simulink model "rolling_contact_36_example"  (R2026b)
settings: Solver=VariableStepAuto  StopTime=5
undefined symbols (not defined in the file): f_rr, k_gx, k_gy, k_x, m_wheel, miu_p, miu_s, mu_slide, mu_stick, omega_rr_eps, r_wheel, sgn, v_gx_max, v_gy_max, vLimit, X, Y, Z
libraries: nesl_utility x225, sm_lib x156, simulink x146, simulink_extras x36
(part 6 of 11)

== system rolling_contact_36_example/36-Point Sliding Contact Model/Body Contact 8 ==
  note: Planar Ground Interaction Model
  " Body Actuator" : nesl_utility/Simulink-PS Converter  PhysicalDomain=network_engine_domain  SubClassName=ps_input  LeftPortType=input  RightPortType=output  PseudoPeriodic=off  Frequencies=[]  NoiseDistribution=none  NoiseParameters=[]  Unit=N  AffineConversion=off  FilteringAndDerivatives=zero  SimscapeFilterOrder=1  InputFilterTimeConstant=.001  UdotUserProvided=0
  " Body Actuator1" : nesl_utility/Simulink-PS Converter  PhysicalDomain=network_engine_domain  SubClassName=ps_input  LeftPortType=input  RightPortType=output  PseudoPeriodic=off  Frequencies=[]  NoiseDistribution=none  NoiseParameters=[]  Unit=N  AffineConversion=off  FilteringAndDerivatives=zero  SimscapeFilterOrder=1  InputFilterTimeConstant=.001  UdotUserProvided=0
  External Force and Torque : sm_lib/Forces and Torques/External Force and Torque  EnableForceX=on  EnableForceY=on  EnableForceZ=off  EnableForce=off  ForceResolutionFrame=World  EnableTorqueX=off  EnableTorqueY=off  EnableTorqueZ=off  EnableTorque=off  TorqueResolutionFrame=AttachedFrame
  Frame Sensor : sm_lib/Frames and Transforms/Transform Sensor  ObservationFrame=World  ExpressedInFrame=World  RotationSequence=XYX  SenseAngle=off  SenseAxis=off  SenseQ=off  SenseR=off  SenseRotationSequence=off  SenseOmegaX=off  SenseOmegaY=off  SenseOmegaZ=off  SenseOmega=off  SenseQDot=off  SenseRDot=off  SenseRotationSequenceDot=off  SenseAlphaX=off  SenseAlphaY=off  SenseAlphaZ=off  SenseAlpha=off  SenseQDDot=off  SenseRDDot=off  SenseX=on  SenseY=on  SenseZ=off  SenseXYZ=off  SenseRad=off  SenseAzim=off  SenseDist=off  SenseInc=off  SenseXDot=on  SenseYDot=on  SenseZDot=off  SenseXYZDot=off  SenseRadDot=off  SenseAzimDot=off  SenseDistDot=off  SenseIncDot=off  SenseXDDot=off  SenseYDDot=off  SenseZDDot=off  SenseXYZDDot=off  SenseRadDDot=off  SenseAzimDDot=off  SenseDistDDot=off  SenseIncDDot=off
  Ground Friction Model : Subsystem
  PS-Simulink Converter : nesl_utility/PS-Simulink Converter  PhysicalDomain=network_engine_domain  SubClassName=ps_output  LeftPortType=input  RightPortType=output  PseudoPeriodic=off  Frequencies=[]  VectorFormat=1-D array  Unit=m  AffineConversion=off
  PS-Simulink Converter1 : nesl_utility/PS-Simulink Converter  PhysicalDomain=network_engine_domain  SubClassName=ps_output  LeftPortType=input  RightPortType=output  PseudoPeriodic=off  Frequencies=[]  VectorFormat=1-D array  Unit=m  AffineConversion=off
  PS-Simulink Converter2 : nesl_utility/PS-Simulink Converter  PhysicalDomain=network_engine_domain  SubClassName=ps_output  LeftPortType=input  RightPortType=output  PseudoPeriodic=off  Frequencies=[]  VectorFormat=1-D array  Unit=m/s  AffineConversion=off
  PS-Simulink Converter3 : nesl_utility/PS-Simulink Converter  PhysicalDomain=network_engine_domain  SubClassName=ps_output  LeftPortType=input  RightPortType=output  PseudoPeriodic=off  Frequencies=[]  VectorFormat=1-D array  Unit=m/s  AffineConversion=off
  Sum : Sum  Inputs=-+|
  Terminator : Terminator
  World Frame : sm_lib/Frames and Transforms/World Frame
  contact sensor : simulink/Logic and Bit Operations/Compare To Zero  relop=<=  OutDataTypeStr=boolean
  yGround : Constant  Value=0
  F : PMIOPort  Side=Left
  Fx patch [N] : Outport
  Fy patch [N] : Outport  Port=2
  wires:
  Ground Friction Model/3(Stiction!) -> Terminator/1
  Ground Friction Model/2(Fx_Friction [N]) -> " Body Actuator"/1, Fx patch [N]/1
  Ground Friction Model/1(Fy_Ground[N]) -> " Body Actuator1"/1, Fy patch [N]/1
  contact sensor/1 -> Ground Friction Model/Enable
  yGround/1 -> Sum/1
  Sum/1 -> Ground Friction Model/1(dy [m]), contact sensor/1
  PS-Simulink Converter1/1 -> Sum/2
  PS-Simulink Converter3/1 -> Ground Friction Model/2(vy [m/s])
  PS-Simulink Converter/1 -> Ground Friction Model/3(x [m])
  PS-Simulink Converter2/1 -> Ground Friction Model/4(vx [m/s])
  connections:
  External Force and Torque/LConn1 -- " Body Actuator"/RConn1
  External Force and Torque/LConn2 -- " Body Actuator1"/RConn1
  F/RConn1 -- Frame Sensor/RConn1 -- External Force and Torque/RConn1
  PS-Simulink Converter3/LConn1 -- Frame Sensor/RConn5
  Frame Sensor/RConn2 -- PS-Simulink Converter/LConn1
  PS-Simulink Converter1/LConn1 -- Frame Sensor/RConn3
  PS-Simulink Converter2/LConn1 -- Frame Sensor/RConn4
  World Frame/RConn1 -- Frame Sensor/LConn1

== system rolling_contact_36_example/36-Point Sliding Contact Model/Body Contact 9 ==
  note: Planar Ground Interaction Model
  " Body Actuator" : nesl_utility/Simulink-PS Converter  PhysicalDomain=network_engine_domain  SubClassName=ps_input  LeftPortType=input  RightPortType=output  PseudoPeriodic=off  Frequencies=[]  NoiseDistribution=none  NoiseParameters=[]  Unit=N  AffineConversion=off  FilteringAndDerivatives=zero  SimscapeFilterOrder=1  InputFilterTimeConstant=.001  UdotUserProvided=0
  " Body Actuator1" : nesl_utility/Simulink-PS Converter  PhysicalDomain=network_engine_domain  SubClassName=ps_input  LeftPortType=input  RightPortType=output  PseudoPeriodic=off  Frequencies=[]  NoiseDistribution=none  NoiseParameters=[]  Unit=N  AffineConversion=off  FilteringAndDerivatives=zero  SimscapeFilterOrder=1  InputFilterTimeConstant=.001  UdotUserProvided=0
  External Force and Torque : sm_lib/Forces and Torques/External Force and Torque  EnableForceX=on  EnableForceY=on  EnableForceZ=off  EnableForce=off  ForceResolutionFrame=World  EnableTorqueX=off  EnableTorqueY=off  EnableTorqueZ=off  EnableTorque=off  TorqueResolutionFrame=AttachedFrame
  Frame Sensor : sm_lib/Frames and Transforms/Transform Sensor  ObservationFrame=World  ExpressedInFrame=World  RotationSequence=XYX  SenseAngle=off  SenseAxis=off  SenseQ=off  SenseR=off  SenseRotationSequence=off  SenseOmegaX=off  SenseOmegaY=off  SenseOmegaZ=off  SenseOmega=off  SenseQDot=off  SenseRDot=off  SenseRotationSequenceDot=off  SenseAlphaX=off  SenseAlphaY=off  SenseAlphaZ=off  SenseAlpha=off  SenseQDDot=off  SenseRDDot=off  SenseX=on  SenseY=on  SenseZ=off  SenseXYZ=off  SenseRad=off  SenseAzim=off  SenseDist=off  SenseInc=off  SenseXDot=on  SenseYDot=on  SenseZDot=off  SenseXYZDot=off  SenseRadDot=off  SenseAzimDot=off  SenseDistDot=off  SenseIncDot=off  SenseXDDot=off  SenseYDDot=off  SenseZDDot=off  SenseXYZDDot=off  SenseRadDDot=off  SenseAzimDDot=off  SenseDistDDot=off  SenseIncDDot=off
  Ground Friction Model : Subsystem
  PS-Simulink Converter : nesl_utility/PS-Simulink Converter  PhysicalDomain=network_engine_domain  SubClassName=ps_output  LeftPortType=input  RightPortType=output  PseudoPeriodic=off  Frequencies=[]  VectorFormat=1-D array  Unit=m  AffineConversion=off
  PS-Simulink Converter1 : nesl_utility/PS-Simulink Converter  PhysicalDomain=network_engine_domain  SubClassName=ps_output  LeftPortType=input  RightPortType=output  PseudoPeriodic=off  Frequencies=[]  VectorFormat=1-D array  Unit=m  AffineConversion=off
  PS-Simulink Converter2 : nesl_utility/PS-Simulink Converter  PhysicalDomain=network_engine_domain  SubClassName=ps_output  LeftPortType=input  RightPortType=output  PseudoPeriodic=off  Frequencies=[]  VectorFormat=1-D array  Unit=m/s  AffineConversion=off
  PS-Simulink Converter3 : nesl_utility/PS-Simulink Converter  PhysicalDomain=network_engine_domain  SubClassName=ps_output  LeftPortType=input  RightPortType=output  PseudoPeriodic=off  Frequencies=[]  VectorFormat=1-D array  Unit=m/s  AffineConversion=off
  Sum : Sum  Inputs=-+|
  Terminator : Terminator
  World Frame : sm_lib/Frames and Transforms/World Frame
  contact sensor : simulink/Logic and Bit Operations/Compare To Zero  relop=<=  OutDataTypeStr=boolean
  yGround : Constant  Value=0
  F : PMIOPort  Side=Left
  Fx patch [N] : Outport
  Fy patch [N] : Outport  Port=2
  wires:
  PS-Simulink Converter2/1 -> Ground Friction Model/4(vx [m/s])
  PS-Simulink Converter/1 -> Ground Friction Model/3(x [m])
  PS-Simulink Converter3/1 -> Ground Friction Model/2(vy [m/s])
  PS-Simulink Converter1/1 -> Sum/2
  Sum/1 -> contact sensor/1, Ground Friction Model/1(dy [m])
  yGround/1 -> Sum/1
  contact sensor/1 -> Ground Friction Model/Enable
  Ground Friction Model/1(Fy_Ground[N]) -> " Body Actuator1"/1, Fy patch [N]/1
  Ground Friction Model/2(Fx_Friction [N]) -> " Body Actuator"/1, Fx patch [N]/1
  Ground Friction Model/3(Stiction!) -> Terminator/1
  connections:
  World Frame/RConn1 -- Frame Sensor/LConn1
  PS-Simulink Converter2/LConn1 -- Frame Sensor/RConn4
  PS-Simulink Converter1/LConn1 -- Frame Sensor/RConn3
  Frame Sensor/RConn2 -- PS-Simulink Converter/LConn1
  PS-Simulink Converter3/LConn1 -- Frame Sensor/RConn5
  External Force and Torque/RConn1 -- Frame Sensor/RConn1 -- F/RConn1
  External Force and Torque/LConn2 -- " Body Actuator1"/RConn1
  External Force and Torque/LConn1 -- " Body Actuator"/RConn1

== system rolling_contact_36_example/Rolling Contact Model/Rolling Resistance Model ==
  Fy [N] : Inport
  wheel speed [rad/s] : Inport  Port=2
  Contact! : EnablePort
  Input Mux : Mux  Inputs=2
  Rolling Resistance Law : Fcn  Expr=-f_rr * u(2) * r_wheel * tanh(u(1) / omega_rr_eps)
  tau_rr [N*m] : Outport
  wires:
  wheel speed [rad/s]/1 -> Input Mux/1
  Fy [N]/1 -> Input Mux/2
  Rolling Resistance Law/1 -> tau_rr [N*m]/1
  Input Mux/1 -> Rolling Resistance Law/1

== system rolling_contact_36_example/Rolling Contact Model/Slip Resistance Model ==
  note: Normal Contact Force
  note: Slip Resistance Force
  note: Peak Slip Ratio (lambda*)
  dy [m] : Inport
  vy [m/s] : Inport  Port=2
  slip ratio : Inport  Port=3
  Contact! : EnablePort  StatesWhenEnabling=reset
  Characteristic Slip Ratio : Fcn  Expr=(3 * miu_p * u(2))/(2 * (u(1)^2 + 0.000000000001) * k_x)
  Constant : Constant  Value=k_x
  Constant1 : Constant  Value=miu_p
  Constant2 : Constant  Value=miu_s
  Gain : Gain  Gain=-r_wheel
  Gain3 : Gain  Gain=pi/4 * E * 1
  Gain4 : Gain  Gain=1/v_gy_max
  Longitudinal Brush Force : MATLAB Function  TreatAsAtomicUnit=on
  Mux : Mux  Inputs=2
  Mux1 : Mux  Inputs=2
  Sqrt : Sqrt
  Y-Axis Ground Force : Fcn  Expr=- u(1) * (1-u(2)) * (u(2)<1)
  Fy_Ground[N] : Outport  OutputWhenDisabled=reset  InitialOutput=0
      settings: AttributesFormatString=initial = '%<InitialOutput>'\nwhen disabled = '%<OutputWhenDisabled>'
  Fx_Friction [N] : Outport  Port=2  OutputWhenDisabled=reset  InitialOutput=0
      settings: AttributesFormatString=initial = '%<InitialOutput>'\nwhen\ndisabled\n'%<OutputWhenDisabled>'
  wires:
  Gain4/1 -> Mux/2
  dy [m]/1 -> Gain3/1, Gain/1  "displacement"
  Mux/1 -> Y-Axis Ground Force/1
  vy [m/s]/1 -> Gain4/1
  Gain3/1 -> Mux/1
  Gain/1 -> Sqrt/1
  Sqrt/1 -> Longitudinal Brush Force/3(a), Mux1/1  "1/2 contact width (a)"
  Mux1/1 -> Characteristic Slip Ratio/1
  Y-Axis Ground Force/1 -> Fy_Ground[N]/1, Longitudinal Brush Force/4(Fy), Mux1/2
  slip ratio/1 -> Longitudinal Brush Force/1(lamda)
  Characteristic Slip Ratio/1 -> Longitudinal Brush Force/2(lamda_c)
  Constant/1 -> Longitudinal Brush Force/5(k_x)
  Constant1/1 -> Longitudinal Brush Force/6(miu_p)
  Constant2/1 -> Longitudinal Brush Force/7(miu_s)
  Longitudinal Brush Force/1(y) -> Fx_Friction [N]/1

== system rolling_contact_36_example/36-Point Sliding Contact Model/Body Contact /Ground Friction Model ==
  note: Vertical Ground Stiction Model
  note: Horizontal Ground Friction Model
  dy [m] : Inport
  vy [m/s] : Inport  Port=2
  x [m] : Inport  Port=3
  vx [m/s] : Inport  Port=4
  Contact! : EnablePort  StatesWhenEnabling=reset
  Data Type Conversion : DataTypeConversion  OutDataTypeStr=double  SaturateOnIntegerOverflow=off  RndMeth=Floor
  Friction Switch : Subsystem
  Gain3 : Gain  Gain=k_gy
  Gain4 : Gain  Gain=1/v_gy_max
  Logical Operator : Logic  Operator=NOT  AllPortsSameDT=off  OutDataTypeStr=boolean
  Mux1 : Mux  Inputs=2
  Sum1 : Sum
  X-Axis Kinetic Friction Model : Subsystem
  X-Axis Static Friction Model : Subsystem
  Y-Axis Ground Force : Fcn  Expr="- u(1)  *  (1-u(2)) * (u(2)<1)"
  Fy_Ground[N] : Outport  OutputWhenDisabled=reset  InitialOutput=0
      settings: AttributesFormatString=initial = '%<InitialOutput>'\nwhen disabled = '%<OutputWhenDisabled>'
  Fx_Friction [N] : Outport  Port=2  OutputWhenDisabled=reset  InitialOutput=0
      settings: AttributesFormatString=initial = '%<InitialOutput>'\nwhen\ndisabled\n'%<OutputWhenDisabled>'
  Stiction! : Outport  Port=3  OutputWhenDisabled=reset  InitialOutput=0
      settings: AttributesFormatString=initial = '%<InitialOutput>'\nwhen\ndisabled\n'%<OutputWhenDisabled>'
  wires:
  Gain4/1 -> Mux1/2
  Gain3/1 -> Mux1/1
  Mux1/1 -> Y-Axis Ground Force/1
  Data Type Conversion/1 -> Stiction!/1
  Logical Operator/1 -> X-Axis Kinetic Friction Model/Enable
  X-Axis Kinetic Friction Model/2(Stiction!) -> Friction Switch/2(Stick!)
  X-Axis Static Friction Model/2(Sliding!) -> Friction Switch/1(Slide!)
  Friction Switch/1(Stiction) -> Data Type Conversion/1, Logical Operator/1, X-Axis Static Friction Model/Enable
  Sum1/1 -> Fx_Friction [N]/1
  X-Axis Static Friction Model/1(F_Stick [N]) -> Sum1/1
  X-Axis Kinetic Friction Model/3(F_Slide [N]) -> Sum1/2
  X-Axis Kinetic Friction Model/1(posFP [m]) -> X-Axis Static Friction Model/4(posFP [m])
  vx [m/s]/1 -> X-Axis Kinetic Friction Model/2(vel [m/s]), X-Axis Static Friction Model/3(vel [m/s])
  x [m]/1 -> X-Axis Kinetic Friction Model/1(pos [m]), X-Axis Static Friction Model/2(pos [m])
  vy [m/s]/1 -> Gain4/1
  dy [m]/1 -> Gain3/1
  Y-Axis Ground Force/1 -> Fy_Ground[N]/1, X-Axis Kinetic Friction Model/3(F_Normal [N]), X-Axis Static Friction Model/1(F_Normal [N])

== system rolling_contact_36_example/36-Point Sliding Contact Model/Body Contact 1/Ground Friction Model ==
  note: Horizontal Ground Friction Model
  note: Vertical Ground Stiction Model
  dy [m] : Inport
  vy [m/s] : Inport  Port=2
  x [m] : Inport  Port=3
  vx [m/s] : Inport  Port=4
  Contact! : EnablePort  StatesWhenEnabling=reset
  Data Type Conversion : DataTypeConversion  OutDataTypeStr=double  SaturateOnIntegerOverflow=off  RndMeth=Floor
  Friction Switch : Subsystem
  Gain3 : Gain  Gain=k_gy
  Gain4 : Gain  Gain=1/v_gy_max
  Logical Operator : Logic  Operator=NOT  AllPortsSameDT=off  OutDataTypeStr=boolean
  Mux1 : Mux  Inputs=2
  Sum1 : Sum
  X-Axis Kinetic Friction Model : Subsystem
  X-Axis Static Friction Model : Subsystem
  Y-Axis Ground Force : Fcn  Expr="- u(1)  *  (1-u(2)) * (u(2)<1)"
  Fy_Ground[N] : Outport  OutputWhenDisabled=reset  InitialOutput=0
      settings: AttributesFormatString=initial = '%<InitialOutput>'\nwhen disabled = '%<OutputWhenDisabled>'
  Fx_Friction [N] : Outport  Port=2  OutputWhenDisabled=reset  InitialOutput=0
      settings: AttributesFormatString=initial = '%<InitialOutput>'\nwhen\ndisabled\n'%<OutputWhenDisabled>'
  Stiction! : Outport  Port=3  OutputWhenDisabled=reset  InitialOutput=0
      settings: AttributesFormatString=initial = '%<InitialOutput>'\nwhen\ndisabled\n'%<OutputWhenDisabled>'
  wires:
  Y-Axis Ground Force/1 -> X-Axis Static Friction Model/1(F_Normal [N]), X-Axis Kinetic Friction Model/3(F_Normal [N]), Fy_Ground[N]/1
  dy [m]/1 -> Gain3/1
  vy [m/s]/1 -> Gain4/1
  x [m]/1 -> X-Axis Static Friction Model/2(pos [m]), X-Axis Kinetic Friction Model/1(pos [m])
  vx [m/s]/1 -> X-Axis Static Friction Model/3(vel [m/s]), X-Axis Kinetic Friction Model/2(vel [m/s])
  X-Axis Kinetic Friction Model/1(posFP [m]) -> X-Axis Static Friction Model/4(posFP [m])
  X-Axis Kinetic Friction Model/3(F_Slide [N]) -> Sum1/2
  X-Axis Static Friction Model/1(F_Stick [N]) -> Sum1/1
  Sum1/1 -> Fx_Friction [N]/1
  Friction Switch/1(Stiction) -> X-Axis Static Friction Model/Enable, Logical Operator/1, Data Type Conversion/1
  X-Axis Static Friction Model/2(Sliding!) -> Friction Switch/1(Slide!)
  X-Axis Kinetic Friction Model/2(Stiction!) -> Friction Switch/2(Stick!)
  Logical Operator/1 -> X-Axis Kinetic Friction Model/Enable
  Data Type Conversion/1 -> Stiction!/1
  Mux1/1 -> Y-Axis Ground Force/1
  Gain3/1 -> Mux1/1
  Gain4/1 -> Mux1/2

== system rolling_contact_36_example/36-Point Sliding Contact Model/Body Contact 10/Ground Friction Model ==
  note: Vertical Ground Stiction Model
  note: Horizontal Ground Friction Model
  dy [m] : Inport
  vy [m/s] : Inport  Port=2
  x [m] : Inport  Port=3
  vx [m/s] : Inport  Port=4
  Contact! : EnablePort  StatesWhenEnabling=reset
  Data Type Conversion : DataTypeConversion  OutDataTypeStr=double  SaturateOnIntegerOverflow=off  RndMeth=Floor
  Friction Switch : Subsystem
  Gain3 : Gain  Gain=k_gy
  Gain4 : Gain  Gain=1/v_gy_max
  Logical Operator : Logic  Operator=NOT  AllPortsSameDT=off  OutDataTypeStr=boolean
  Mux1 : Mux  Inputs=2
  Sum1 : Sum
  X-Axis Kinetic Friction Model : Subsystem
  X-Axis Static Friction Model : Subsystem
  Y-Axis Ground Force : Fcn  Expr="- u(1)  *  (1-u(2)) * (u(2)<1)"
  Fy_Ground[N] : Outport  OutputWhenDisabled=reset  InitialOutput=0
      settings: AttributesFormatString=initial = '%<InitialOutput>'\nwhen disabled = '%<OutputWhenDisabled>'
  Fx_Friction [N] : Outport  Port=2  OutputWhenDisabled=reset  InitialOutput=0
      settings: AttributesFormatString=initial = '%<InitialOutput>'\nwhen\ndisabled\n'%<OutputWhenDisabled>'
  Stiction! : Outport  Port=3  OutputWhenDisabled=reset  InitialOutput=0
      settings: AttributesFormatString=initial = '%<InitialOutput>'\nwhen\ndisabled\n'%<OutputWhenDisabled>'
  wires:
  Gain4/1 -> Mux1/2
  Gain3/1 -> Mux1/1
  Mux1/1 -> Y-Axis Ground Force/1
  Data Type Conversion/1 -> Stiction!/1
  Logical Operator/1 -> X-Axis Kinetic Friction Model/Enable
  X-Axis Kinetic Friction Model/2(Stiction!) -> Friction Switch/2(Stick!)
  X-Axis Static Friction Model/2(Sliding!) -> Friction Switch/1(Slide!)
  Friction Switch/1(Stiction) -> Data Type Conversion/1, Logical Operator/1, X-Axis Static Friction Model/Enable
  Sum1/1 -> Fx_Friction [N]/1
  X-Axis Static Friction Model/1(F_Stick [N]) -> Sum1/1
  X-Axis Kinetic Friction Model/3(F_Slide [N]) -> Sum1/2
  X-Axis Kinetic Friction Model/1(posFP [m]) -> X-Axis Static Friction Model/4(posFP [m])
  vx [m/s]/1 -> X-Axis Kinetic Friction Model/2(vel [m/s]), X-Axis Static Friction Model/3(vel [m/s])
  x [m]/1 -> X-Axis Kinetic Friction Model/1(pos [m]), X-Axis Static Friction Model/2(pos [m])
  vy [m/s]/1 -> Gain4/1
  dy [m]/1 -> Gain3/1
  Y-Axis Ground Force/1 -> Fy_Ground[N]/1, X-Axis Kinetic Friction Model/3(F_Normal [N]), X-Axis Static Friction Model/1(F_Normal [N])

== system rolling_contact_36_example/36-Point Sliding Contact Model/Body Contact 11/Ground Friction Model ==
  note: Horizontal Ground Friction Model
  note: Vertical Ground Stiction Model
  dy [m] : Inport
  vy [m/s] : Inport  Port=2
  x [m] : Inport  Port=3
  vx [m/s] : Inport  Port=4
  Contact! : EnablePort  StatesWhenEnabling=reset
  Data Type Conversion : DataTypeConversion  OutDataTypeStr=double  SaturateOnIntegerOverflow=off  RndMeth=Floor
  Friction Switch : Subsystem
  Gain3 : Gain  Gain=k_gy
  Gain4 : Gain  Gain=1/v_gy_max
  Logical Operator : Logic  Operator=NOT  AllPortsSameDT=off  OutDataTypeStr=boolean
  Mux1 : Mux  Inputs=2
  Sum1 : Sum
  X-Axis Kinetic Friction Model : Subsystem
  X-Axis Static Friction Model : Subsystem
  Y-Axis Ground Force : Fcn  Expr="- u(1)  *  (1-u(2)) * (u(2)<1)"
  Fy_Ground[N] : Outport  OutputWhenDisabled=reset  InitialOutput=0
      settings: AttributesFormatString=initial = '%<InitialOutput>'\nwhen disabled = '%<OutputWhenDisabled>'
  Fx_Friction [N] : Outport  Port=2  OutputWhenDisabled=reset  InitialOutput=0
      settings: AttributesFormatString=initial = '%<InitialOutput>'\nwhen\ndisabled\n'%<OutputWhenDisabled>'
  Stiction! : Outport  Port=3  OutputWhenDisabled=reset  InitialOutput=0
      settings: AttributesFormatString=initial = '%<InitialOutput>'\nwhen\ndisabled\n'%<OutputWhenDisabled>'
  wires:
  Y-Axis Ground Force/1 -> X-Axis Static Friction Model/1(F_Normal [N]), X-Axis Kinetic Friction Model/3(F_Normal [N]), Fy_Ground[N]/1
  dy [m]/1 -> Gain3/1
  vy [m/s]/1 -> Gain4/1
  x [m]/1 -> X-Axis Static Friction Model/2(pos [m]), X-Axis Kinetic Friction Model/1(pos [m])
  vx [m/s]/1 -> X-Axis Static Friction Model/3(vel [m/s]), X-Axis Kinetic Friction Model/2(vel [m/s])
  X-Axis Kinetic Friction Model/1(posFP [m]) -> X-Axis Static Friction Model/4(posFP [m])
  X-Axis Kinetic Friction Model/3(F_Slide [N]) -> Sum1/2
  X-Axis Static Friction Model/1(F_Stick [N]) -> Sum1/1
  Sum1/1 -> Fx_Friction [N]/1
  Friction Switch/1(Stiction) -> X-Axis Static Friction Model/Enable, Logical Operator/1, Data Type Conversion/1
  X-Axis Static Friction Model/2(Sliding!) -> Friction Switch/1(Slide!)
  X-Axis Kinetic Friction Model/2(Stiction!) -> Friction Switch/2(Stick!)
  Logical Operator/1 -> X-Axis Kinetic Friction Model/Enable
  Data Type Conversion/1 -> Stiction!/1
  Mux1/1 -> Y-Axis Ground Force/1
  Gain3/1 -> Mux1/1
  Gain4/1 -> Mux1/2

== system rolling_contact_36_example/36-Point Sliding Contact Model/Body Contact 12/Ground Friction Model ==
  note: Vertical Ground Stiction Model
  note: Horizontal Ground Friction Model
  dy [m] : Inport
  vy [m/s] : Inport  Port=2
  x [m] : Inport  Port=3
  vx [m/s] : Inport  Port=4
  Contact! : EnablePort  StatesWhenEnabling=reset
  Data Type Conversion : DataTypeConversion  OutDataTypeStr=double  SaturateOnIntegerOverflow=off  RndMeth=Floor
  Friction Switch : Subsystem
  Gain3 : Gain  Gain=k_gy
  Gain4 : Gain  Gain=1/v_gy_max
  Logical Operator : Logic  Operator=NOT  AllPortsSameDT=off  OutDataTypeStr=boolean
  Mux1 : Mux  Inputs=2
  Sum1 : Sum
  X-Axis Kinetic Friction Model : Subsystem
  X-Axis Static Friction Model : Subsystem
  Y-Axis Ground Force : Fcn  Expr="- u(1)  *  (1-u(2)) * (u(2)<1)"
  Fy_Ground[N] : Outport  OutputWhenDisabled=reset  InitialOutput=0
      settings: AttributesFormatString=initial = '%<InitialOutput>'\nwhen disabled = '%<OutputWhenDisabled>'
  Fx_Friction [N] : Outport  Port=2  OutputWhenDisabled=reset  InitialOutput=0
      settings: AttributesFormatString=initial = '%<InitialOutput>'\nwhen\ndisabled\n'%<OutputWhenDisabled>'
  Stiction! : Outport  Port=3  OutputWhenDisabled=reset  InitialOutput=0
      settings: AttributesFormatString=initial = '%<InitialOutput>'\nwhen\ndisabled\n'%<OutputWhenDisabled>'
  wires:
  Gain4/1 -> Mux1/2
  Gain3/1 -> Mux1/1
  Mux1/1 -> Y-Axis Ground Force/1
  Data Type Conversion/1 -> Stiction!/1
  Logical Operator/1 -> X-Axis Kinetic Friction Model/Enable
  X-Axis Kinetic Friction Model/2(Stiction!) -> Friction Switch/2(Stick!)
  X-Axis Static Friction Model/2(Sliding!) -> Friction Switch/1(Slide!)
  Friction Switch/1(Stiction) -> Data Type Conversion/1, Logical Operator/1, X-Axis Static Friction Model/Enable
  Sum1/1 -> Fx_Friction [N]/1
  X-Axis Static Friction Model/1(F_Stick [N]) -> Sum1/1
  X-Axis Kinetic Friction Model/3(F_Slide [N]) -> Sum1/2
  X-Axis Kinetic Friction Model/1(posFP [m]) -> X-Axis Static Friction Model/4(posFP [m])
  vx [m/s]/1 -> X-Axis Kinetic Friction Model/2(vel [m/s]), X-Axis Static Friction Model/3(vel [m/s])
  x [m]/1 -> X-Axis Kinetic Friction Model/1(pos [m]), X-Axis Static Friction Model/2(pos [m])
  vy [m/s]/1 -> Gain4/1
  dy [m]/1 -> Gain3/1
  Y-Axis Ground Force/1 -> Fy_Ground[N]/1, X-Axis Kinetic Friction Model/3(F_Normal [N]), X-Axis Static Friction Model/1(F_Normal [N])

== system rolling_contact_36_example/36-Point Sliding Contact Model/Body Contact 13/Ground Friction Model ==
  note: Horizontal Ground Friction Model
  note: Vertical Ground Stiction Model
  dy [m] : Inport
  vy [m/s] : Inport  Port=2
  x [m] : Inport  Port=3
  vx [m/s] : Inport  Port=4
  Contact! : EnablePort  StatesWhenEnabling=reset
  Data Type Conversion : DataTypeConversion  OutDataTypeStr=double  SaturateOnIntegerOverflow=off  RndMeth=Floor
  Friction Switch : Subsystem
  Gain3 : Gain  Gain=k_gy
  Gain4 : Gain  Gain=1/v_gy_max
  Logical Operator : Logic  Operator=NOT  AllPortsSameDT=off  OutDataTypeStr=boolean
  Mux1 : Mux  Inputs=2
  Sum1 : Sum
  X-Axis Kinetic Friction Model : Subsystem
  X-Axis Static Friction Model : Subsystem
  Y-Axis Ground Force : Fcn  Expr="- u(1)  *  (1-u(2)) * (u(2)<1)"
  Fy_Ground[N] : Outport  OutputWhenDisabled=reset  InitialOutput=0
      settings: AttributesFormatString=initial = '%<InitialOutput>'\nwhen disabled = '%<OutputWhenDisabled>'
  Fx_Friction [N] : Outport  Port=2  OutputWhenDisabled=reset  InitialOutput=0
      settings: AttributesFormatString=initial = '%<InitialOutput>'\nwhen\ndisabled\n'%<OutputWhenDisabled>'
  Stiction! : Outport  Port=3  OutputWhenDisabled=reset  InitialOutput=0
      settings: AttributesFormatString=initial = '%<InitialOutput>'\nwhen\ndisabled\n'%<OutputWhenDisabled>'
  wires:
  Y-Axis Ground Force/1 -> X-Axis Static Friction Model/1(F_Normal [N]), X-Axis Kinetic Friction Model/3(F_Normal [N]), Fy_Ground[N]/1
  dy [m]/1 -> Gain3/1
  vy [m/s]/1 -> Gain4/1
  x [m]/1 -> X-Axis Static Friction Model/2(pos [m]), X-Axis Kinetic Friction Model/1(pos [m])
  vx [m/s]/1 -> X-Axis Static Friction Model/3(vel [m/s]), X-Axis Kinetic Friction Model/2(vel [m/s])
  X-Axis Kinetic Friction Model/1(posFP [m]) -> X-Axis Static Friction Model/4(posFP [m])
  X-Axis Kinetic Friction Model/3(F_Slide [N]) -> Sum1/2
  X-Axis Static Friction Model/1(F_Stick [N]) -> Sum1/1
  Sum1/1 -> Fx_Friction [N]/1
  Friction Switch/1(Stiction) -> X-Axis Static Friction Model/Enable, Logical Operator/1, Data Type Conversion/1
  X-Axis Static Friction Model/2(Sliding!) -> Friction Switch/1(Slide!)
  X-Axis Kinetic Friction Model/2(Stiction!) -> Friction Switch/2(Stick!)
  Logical Operator/1 -> X-Axis Kinetic Friction Model/Enable
  Data Type Conversion/1 -> Stiction!/1
  Mux1/1 -> Y-Axis Ground Force/1
  Gain3/1 -> Mux1/1
  Gain4/1 -> Mux1/2

== system rolling_contact_36_example/36-Point Sliding Contact Model/Body Contact 14/Ground Friction Model ==
  note: Vertical Ground Stiction Model
  note: Horizontal Ground Friction Model
  dy [m] : Inport
  vy [m/s] : Inport  Port=2
  x [m] : Inport  Port=3
  vx [m/s] : Inport  Port=4
  Contact! : EnablePort  StatesWhenEnabling=reset
  Data Type Conversion : DataTypeConversion  OutDataTypeStr=double  SaturateOnIntegerOverflow=off  RndMeth=Floor
  Friction Switch : Subsystem
  Gain3 : Gain  Gain=k_gy
  Gain4 : Gain  Gain=1/v_gy_max
  Logical Operator : Logic  Operator=NOT  AllPortsSameDT=off  OutDataTypeStr=boolean
  Mux1 : Mux  Inputs=2
  Sum1 : Sum
  X-Axis Kinetic Friction Model : Subsystem
  X-Axis Static Friction Model : Subsystem
  Y-Axis Ground Force : Fcn  Expr="- u(1)  *  (1-u(2)) * (u(2)<1)"
  Fy_Ground[N] : Outport  OutputWhenDisabled=reset  InitialOutput=0
      settings: AttributesFormatString=initial = '%<InitialOutput>'\nwhen disabled = '%<OutputWhenDisabled>'
  Fx_Friction [N] : Outport  Port=2  OutputWhenDisabled=reset  InitialOutput=0
      settings: AttributesFormatString=initial = '%<InitialOutput>'\nwhen\ndisabled\n'%<OutputWhenDisabled>'
  Stiction! : Outport  Port=3  OutputWhenDisabled=reset  InitialOutput=0
      settings: AttributesFormatString=initial = '%<InitialOutput>'\nwhen\ndisabled\n'%<OutputWhenDisabled>'
  wires:
  Gain4/1 -> Mux1/2
  Gain3/1 -> Mux1/1
  Mux1/1 -> Y-Axis Ground Force/1
  Data Type Conversion/1 -> Stiction!/1
  Logical Operator/1 -> X-Axis Kinetic Friction Model/Enable
  X-Axis Kinetic Friction Model/2(Stiction!) -> Friction Switch/2(Stick!)
  X-Axis Static Friction Model/2(Sliding!) -> Friction Switch/1(Slide!)
  Friction Switch/1(Stiction) -> Data Type Conversion/1, Logical Operator/1, X-Axis Static Friction Model/Enable
  Sum1/1 -> Fx_Friction [N]/1
  X-Axis Static Friction Model/1(F_Stick [N]) -> Sum1/1
  X-Axis Kinetic Friction Model/3(F_Slide [N]) -> Sum1/2
  X-Axis Kinetic Friction Model/1(posFP [m]) -> X-Axis Static Friction Model/4(posFP [m])
  vx [m/s]/1 -> X-Axis Kinetic Friction Model/2(vel [m/s]), X-Axis Static Friction Model/3(vel [m/s])
  x [m]/1 -> X-Axis Kinetic Friction Model/1(pos [m]), X-Axis Static Friction Model/2(pos [m])
  vy [m/s]/1 -> Gain4/1
  dy [m]/1 -> Gain3/1
  Y-Axis Ground Force/1 -> Fy_Ground[N]/1, X-Axis Kinetic Friction Model/3(F_Normal [N]), X-Axis Static Friction Model/1(F_Normal [N])

== system rolling_contact_36_example/36-Point Sliding Contact Model/Body Contact 15/Ground Friction Model ==
  note: Horizontal Ground Friction Model
  note: Vertical Ground Stiction Model
  dy [m] : Inport
  vy [m/s] : Inport  Port=2
  x [m] : Inport  Port=3
  vx [m/s] : Inport  Port=4
  Contact! : EnablePort  StatesWhenEnabling=reset
  Data Type Conversion : DataTypeConversion  OutDataTypeStr=double  SaturateOnIntegerOverflow=off  RndMeth=Floor
  Friction Switch : Subsystem
  Gain3 : Gain  Gain=k_gy
  Gain4 : Gain  Gain=1/v_gy_max
  Logical Operator : Logic  Operator=NOT  AllPortsSameDT=off  OutDataTypeStr=boolean
  Mux1 : Mux  Inputs=2
  Sum1 : Sum
  X-Axis Kinetic Friction Model : Subsystem
  X-Axis Static Friction Model : Subsystem
  Y-Axis Ground Force : Fcn  Expr="- u(1)  *  (1-u(2)) * (u(2)<1)"
  Fy_Ground[N] : Outport  OutputWhenDisabled=reset  InitialOutput=0
      settings: AttributesFormatString=initial = '%<InitialOutput>'\nwhen disabled = '%<OutputWhenDisabled>'
  Fx_Friction [N] : Outport  Port=2  OutputWhenDisabled=reset  InitialOutput=0
      settings: AttributesFormatString=initial = '%<InitialOutput>'\nwhen\ndisabled\n'%<OutputWhenDisabled>'
  Stiction! : Outport  Port=3  OutputWhenDisabled=reset  InitialOutput=0
      settings: AttributesFormatString=initial = '%<InitialOutput>'\nwhen\ndisabled\n'%<OutputWhenDisabled>'
  wires:
  Y-Axis Ground Force/1 -> X-Axis Static Friction Model/1(F_Normal [N]), X-Axis Kinetic Friction Model/3(F_Normal [N]), Fy_Ground[N]/1
  dy [m]/1 -> Gain3/1
  vy [m/s]/1 -> Gain4/1
  x [m]/1 -> X-Axis Static Friction Model/2(pos [m]), X-Axis Kinetic Friction Model/1(pos [m])
  vx [m/s]/1 -> X-Axis Static Friction Model/3(vel [m/s]), X-Axis Kinetic Friction Model/2(vel [m/s])
  X-Axis Kinetic Friction Model/1(posFP [m]) -> X-Axis Static Friction Model/4(posFP [m])
  X-Axis Kinetic Friction Model/3(F_Slide [N]) -> Sum1/2
  X-Axis Static Friction Model/1(F_Stick [N]) -> Sum1/1
  Sum1/1 -> Fx_Friction [N]/1
  Friction Switch/1(Stiction) -> X-Axis Static Friction Model/Enable, Logical Operator/1, Data Type Conversion/1
  X-Axis Static Friction Model/2(Sliding!) -> Friction Switch/1(Slide!)
  X-Axis Kinetic Friction Model/2(Stiction!) -> Friction Switch/2(Stick!)
  Logical Operator/1 -> X-Axis Kinetic Friction Model/Enable
  Data Type Conversion/1 -> Stiction!/1
  Mux1/1 -> Y-Axis Ground Force/1
  Gain3/1 -> Mux1/1
  Gain4/1 -> Mux1/2

== system rolling_contact_36_example/36-Point Sliding Contact Model/Body Contact 16/Ground Friction Model ==
  note: Vertical Ground Stiction Model
  note: Horizontal Ground Friction Model
  dy [m] : Inport
  vy [m/s] : Inport  Port=2
  x [m] : Inport  Port=3
  vx [m/s] : Inport  Port=4
  Contact! : EnablePort  StatesWhenEnabling=reset
  Data Type Conversion : DataTypeConversion  OutDataTypeStr=double  SaturateOnIntegerOverflow=off  RndMeth=Floor
  Friction Switch : Subsystem
  Gain3 : Gain  Gain=k_gy
  Gain4 : Gain  Gain=1/v_gy_max
  Logical Operator : Logic  Operator=NOT  AllPortsSameDT=off  OutDataTypeStr=boolean
  Mux1 : Mux  Inputs=2
  Sum1 : Sum
  X-Axis Kinetic Friction Model : Subsystem
  X-Axis Static Friction Model : Subsystem
  Y-Axis Ground Force : Fcn  Expr="- u(1)  *  (1-u(2)) * (u(2)<1)"
  Fy_Ground[N] : Outport  OutputWhenDisabled=reset  InitialOutput=0
      settings: AttributesFormatString=initial = '%<InitialOutput>'\nwhen disabled = '%<OutputWhenDisabled>'
  Fx_Friction [N] : Outport  Port=2  OutputWhenDisabled=reset  InitialOutput=0
      settings: AttributesFormatString=initial = '%<InitialOutput>'\nwhen\ndisabled\n'%<OutputWhenDisabled>'
  Stiction! : Outport  Port=3  OutputWhenDisabled=reset  InitialOutput=0
      settings: AttributesFormatString=initial = '%<InitialOutput>'\nwhen\ndisabled\n'%<OutputWhenDisabled>'
  wires:
  Gain4/1 -> Mux1/2
  Gain3/1 -> Mux1/1
  Mux1/1 -> Y-Axis Ground Force/1
  Data Type Conversion/1 -> Stiction!/1
  Logical Operator/1 -> X-Axis Kinetic Friction Model/Enable
  X-Axis Kinetic Friction Model/2(Stiction!) -> Friction Switch/2(Stick!)
  X-Axis Static Friction Model/2(Sliding!) -> Friction Switch/1(Slide!)
  Friction Switch/1(Stiction) -> Data Type Conversion/1, Logical Operator/1, X-Axis Static Friction Model/Enable
  Sum1/1 -> Fx_Friction [N]/1
  X-Axis Static Friction Model/1(F_Stick [N]) -> Sum1/1
  X-Axis Kinetic Friction Model/3(F_Slide [N]) -> Sum1/2
  X-Axis Kinetic Friction Model/1(posFP [m]) -> X-Axis Static Friction Model/4(posFP [m])
  vx [m/s]/1 -> X-Axis Kinetic Friction Model/2(vel [m/s]), X-Axis Static Friction Model/3(vel [m/s])
  x [m]/1 -> X-Axis Kinetic Friction Model/1(pos [m]), X-Axis Static Friction Model/2(pos [m])
  vy [m/s]/1 -> Gain4/1
  dy [m]/1 -> Gain3/1
  Y-Axis Ground Force/1 -> Fy_Ground[N]/1, X-Axis Kinetic Friction Model/3(F_Normal [N]), X-Axis Static Friction Model/1(F_Normal [N])

== system rolling_contact_36_example/36-Point Sliding Contact Model/Body Contact 17/Ground Friction Model ==
  note: Horizontal Ground Friction Model
  note: Vertical Ground Stiction Model
  dy [m] : Inport
  vy [m/s] : Inport  Port=2
  x [m] : Inport  Port=3
  vx [m/s] : Inport  Port=4
  Contact! : EnablePort  StatesWhenEnabling=reset
  Data Type Conversion : DataTypeConversion  OutDataTypeStr=double  SaturateOnIntegerOverflow=off  RndMeth=Floor
  Friction Switch : Subsystem
  Gain3 : Gain  Gain=k_gy
  Gain4 : Gain  Gain=1/v_gy_max
  Logical Operator : Logic  Operator=NOT  AllPortsSameDT=off  OutDataTypeStr=boolean
  Mux1 : Mux  Inputs=2
  Sum1 : Sum
  X-Axis Kinetic Friction Model : Subsystem
  X-Axis Static Friction Model : Subsystem
  Y-Axis Ground Force : Fcn  Expr="- u(1)  *  (1-u(2)) * (u(2)<1)"
  Fy_Ground[N] : Outport  OutputWhenDisabled=reset  InitialOutput=0
      settings: AttributesFormatString=initial = '%<InitialOutput>'\nwhen disabled = '%<OutputWhenDisabled>'
  Fx_Friction [N] : Outport  Port=2  OutputWhenDisabled=reset  InitialOutput=0
      settings: AttributesFormatString=initial = '%<InitialOutput>'\nwhen\ndisabled\n'%<OutputWhenDisabled>'
  Stiction! : Outport  Port=3  OutputWhenDisabled=reset  InitialOutput=0
      settings: AttributesFormatString=initial = '%<InitialOutput>'\nwhen\ndisabled\n'%<OutputWhenDisabled>'
  wires:
  Y-Axis Ground Force/1 -> X-Axis Static Friction Model/1(F_Normal [N]), X-Axis Kinetic Friction Model/3(F_Normal [N]), Fy_Ground[N]/1
  dy [m]/1 -> Gain3/1
  vy [m/s]/1 -> Gain4/1
  x [m]/1 -> X-Axis Static Friction Model/2(pos [m]), X-Axis Kinetic Friction Model/1(pos [m])
  vx [m/s]/1 -> X-Axis Static Friction Model/3(vel [m/s]), X-Axis Kinetic Friction Model/2(vel [m/s])
  X-Axis Kinetic Friction Model/1(posFP [m]) -> X-Axis Static Friction Model/4(posFP [m])
  X-Axis Kinetic Friction Model/3(F_Slide [N]) -> Sum1/2
  X-Axis Static Friction Model/1(F_Stick [N]) -> Sum1/1
  Sum1/1 -> Fx_Friction [N]/1
  Friction Switch/1(Stiction) -> X-Axis Static Friction Model/Enable, Logical Operator/1, Data Type Conversion/1
  X-Axis Static Friction Model/2(Sliding!) -> Friction Switch/1(Slide!)
  X-Axis Kinetic Friction Model/2(Stiction!) -> Friction Switch/2(Stick!)
  Logical Operator/1 -> X-Axis Kinetic Friction Model/Enable
  Data Type Conversion/1 -> Stiction!/1
  Mux1/1 -> Y-Axis Ground Force/1
  Gain3/1 -> Mux1/1
  Gain4/1 -> Mux1/2

== system rolling_contact_36_example/36-Point Sliding Contact Model/Body Contact 18/Ground Friction Model ==
  note: Vertical Ground Stiction Model
  note: Horizontal Ground Friction Model
  dy [m] : Inport
  vy [m/s] : Inport  Port=2
  x [m] : Inport  Port=3
  vx [m/s] : Inport  Port=4
  Contact! : EnablePort  StatesWhenEnabling=reset
  Data Type Conversion : DataTypeConversion  OutDataTypeStr=double  SaturateOnIntegerOverflow=off  RndMeth=Floor
  Friction Switch : Subsystem
  Gain3 : Gain  Gain=k_gy
  Gain4 : Gain  Gain=1/v_gy_max
  Logical Operator : Logic  Operator=NOT  AllPortsSameDT=off  OutDataTypeStr=boolean
  Mux1 : Mux  Inputs=2
  Sum1 : Sum
  X-Axis Kinetic Friction Model : Subsystem
  X-Axis Static Friction Model : Subsystem
  Y-Axis Ground Force : Fcn  Expr="- u(1)  *  (1-u(2)) * (u(2)<1)"
  Fy_Ground[N] : Outport  OutputWhenDisabled=reset  InitialOutput=0
      settings: AttributesFormatString=initial = '%<InitialOutput>'\nwhen disabled = '%<OutputWhenDisabled>'
  Fx_Friction [N] : Outport  Port=2  OutputWhenDisabled=reset  InitialOutput=0
      settings: AttributesFormatString=initial = '%<InitialOutput>'\nwhen\ndisabled\n'%<OutputWhenDisabled>'
  Stiction! : Outport  Port=3  OutputWhenDisabled=reset  InitialOutput=0
      settings: AttributesFormatString=initial = '%<InitialOutput>'\nwhen\ndisabled\n'%<OutputWhenDisabled>'
  wires:
  Gain4/1 -> Mux1/2
  Gain3/1 -> Mux1/1
  Mux1/1 -> Y-Axis Ground Force/1
  Data Type Conversion/1 -> Stiction!/1
  Logical Operator/1 -> X-Axis Kinetic Friction Model/Enable
  X-Axis Kinetic Friction Model/2(Stiction!) -> Friction Switch/2(Stick!)
  X-Axis Static Friction Model/2(Sliding!) -> Friction Switch/1(Slide!)
  Friction Switch/1(Stiction) -> Data Type Conversion/1, Logical Operator/1, X-Axis Static Friction Model/Enable
  Sum1/1 -> Fx_Friction [N]/1
  X-Axis Static Friction Model/1(F_Stick [N]) -> Sum1/1
  X-Axis Kinetic Friction Model/3(F_Slide [N]) -> Sum1/2
  X-Axis Kinetic Friction Model/1(posFP [m]) -> X-Axis Static Friction Model/4(posFP [m])
  vx [m/s]/1 -> X-Axis Kinetic Friction Model/2(vel [m/s]), X-Axis Static Friction Model/3(vel [m/s])
  x [m]/1 -> X-Axis Kinetic Friction Model/1(pos [m]), X-Axis Static Friction Model/2(pos [m])
  vy [m/s]/1 -> Gain4/1
  dy [m]/1 -> Gain3/1
  Y-Axis Ground Force/1 -> Fy_Ground[N]/1, X-Axis Kinetic Friction Model/3(F_Normal [N]), X-Axis Static Friction Model/1(F_Normal [N])

== system rolling_contact_36_example/36-Point Sliding Contact Model/Body Contact 19/Ground Friction Model ==
  note: Horizontal Ground Friction Model
  note: Vertical Ground Stiction Model
  dy [m] : Inport
  vy [m/s] : Inport  Port=2
  x [m] : Inport  Port=3
  vx [m/s] : Inport  Port=4
  Contact! : EnablePort  StatesWhenEnabling=reset
  Data Type Conversion : DataTypeConversion  OutDataTypeStr=double  SaturateOnIntegerOverflow=off  RndMeth=Floor
  Friction Switch : Subsystem
  Gain3 : Gain  Gain=k_gy
  Gain4 : Gain  Gain=1/v_gy_max
  Logical Operator : Logic  Operator=NOT  AllPortsSameDT=off  OutDataTypeStr=boolean
  Mux1 : Mux  Inputs=2
  Sum1 : Sum
  X-Axis Kinetic Friction Model : Subsystem
  X-Axis Static Friction Model : Subsystem
  Y-Axis Ground Force : Fcn  Expr="- u(1)  *  (1-u(2)) * (u(2)<1)"
  Fy_Ground[N] : Outport  OutputWhenDisabled=reset  InitialOutput=0
      settings: AttributesFormatString=initial = '%<InitialOutput>'\nwhen disabled = '%<OutputWhenDisabled>'
  Fx_Friction [N] : Outport  Port=2  OutputWhenDisabled=reset  InitialOutput=0
      settings: AttributesFormatString=initial = '%<InitialOutput>'\nwhen\ndisabled\n'%<OutputWhenDisabled>'
  Stiction! : Outport  Port=3  OutputWhenDisabled=reset  InitialOutput=0
      settings: AttributesFormatString=initial = '%<InitialOutput>'\nwhen\ndisabled\n'%<OutputWhenDisabled>'
  wires:
  Y-Axis Ground Force/1 -> X-Axis Static Friction Model/1(F_Normal [N]), X-Axis Kinetic Friction Model/3(F_Normal [N]), Fy_Ground[N]/1
  dy [m]/1 -> Gain3/1
  vy [m/s]/1 -> Gain4/1
  x [m]/1 -> X-Axis Static Friction Model/2(pos [m]), X-Axis Kinetic Friction Model/1(pos [m])
  vx [m/s]/1 -> X-Axis Static Friction Model/3(vel [m/s]), X-Axis Kinetic Friction Model/2(vel [m/s])
  X-Axis Kinetic Friction Model/1(posFP [m]) -> X-Axis Static Friction Model/4(posFP [m])
  X-Axis Kinetic Friction Model/3(F_Slide [N]) -> Sum1/2
  X-Axis Static Friction Model/1(F_Stick [N]) -> Sum1/1
  Sum1/1 -> Fx_Friction [N]/1
  Friction Switch/1(Stiction) -> X-Axis Static Friction Model/Enable, Logical Operator/1, Data Type Conversion/1
  X-Axis Static Friction Model/2(Sliding!) -> Friction Switch/1(Slide!)
  X-Axis Kinetic Friction Model/2(Stiction!) -> Friction Switch/2(Stick!)
  Logical Operator/1 -> X-Axis Kinetic Friction Model/Enable
  Data Type Conversion/1 -> Stiction!/1
  Mux1/1 -> Y-Axis Ground Force/1
  Gain3/1 -> Mux1/1
  Gain4/1 -> Mux1/2

== system rolling_contact_36_example/36-Point Sliding Contact Model/Body Contact 2/Ground Friction Model ==
  note: Vertical Ground Stiction Model
  note: Horizontal Ground Friction Model
  dy [m] : Inport
  vy [m/s] : Inport  Port=2
  x [m] : Inport  Port=3
  vx [m/s] : Inport  Port=4
  Contact! : EnablePort  StatesWhenEnabling=reset
  Data Type Conversion : DataTypeConversion  OutDataTypeStr=double  SaturateOnIntegerOverflow=off  RndMeth=Floor
  Friction Switch : Subsystem
  Gain3 : Gain  Gain=k_gy
  Gain4 : Gain  Gain=1/v_gy_max
  Logical Operator : Logic  Operator=NOT  AllPortsSameDT=off  OutDataTypeStr=boolean
  Mux1 : Mux  Inputs=2
  Sum1 : Sum
  X-Axis Kinetic Friction Model : Subsystem
  X-Axis Static Friction Model : Subsystem
  Y-Axis Ground Force : Fcn  Expr="- u(1)  *  (1-u(2)) * (u(2)<1)"
  Fy_Ground[N] : Outport  OutputWhenDisabled=reset  InitialOutput=0
      settings: AttributesFormatString=initial = '%<InitialOutput>'\nwhen disabled = '%<OutputWhenDisabled>'
  Fx_Friction [N] : Outport  Port=2  OutputWhenDisabled=reset  InitialOutput=0
      settings: AttributesFormatString=initial = '%<InitialOutput>'\nwhen\ndisabled\n'%<OutputWhenDisabled>'
  Stiction! : Outport  Port=3  OutputWhenDisabled=reset  InitialOutput=0
      settings: AttributesFormatString=initial = '%<InitialOutput>'\nwhen\ndisabled\n'%<OutputWhenDisabled>'
  wires:
  Gain4/1 -> Mux1/2
  Gain3/1 -> Mux1/1
  Mux1/1 -> Y-Axis Ground Force/1
  Data Type Conversion/1 -> Stiction!/1
  Logical Operator/1 -> X-Axis Kinetic Friction Model/Enable
  X-Axis Kinetic Friction Model/2(Stiction!) -> Friction Switch/2(Stick!)
  X-Axis Static Friction Model/2(Sliding!) -> Friction Switch/1(Slide!)
  Friction Switch/1(Stiction) -> Data Type Conversion/1, Logical Operator/1, X-Axis Static Friction Model/Enable
  Sum1/1 -> Fx_Friction [N]/1
  X-Axis Static Friction Model/1(F_Stick [N]) -> Sum1/1
  X-Axis Kinetic Friction Model/3(F_Slide [N]) -> Sum1/2
  X-Axis Kinetic Friction Model/1(posFP [m]) -> X-Axis Static Friction Model/4(posFP [m])
  vx [m/s]/1 -> X-Axis Kinetic Friction Model/2(vel [m/s]), X-Axis Static Friction Model/3(vel [m/s])
  x [m]/1 -> X-Axis Kinetic Friction Model/1(pos [m]), X-Axis Static Friction Model/2(pos [m])
  vy [m/s]/1 -> Gain4/1
  dy [m]/1 -> Gain3/1
  Y-Axis Ground Force/1 -> Fy_Ground[N]/1, X-Axis Kinetic Friction Model/3(F_Normal [N]), X-Axis Static Friction Model/1(F_Normal [N])

== system rolling_contact_36_example/36-Point Sliding Contact Model/Body Contact 20/Ground Friction Model ==
  note: Vertical Ground Stiction Model
  note: Horizontal Ground Friction Model
  dy [m] : Inport
  vy [m/s] : Inport  Port=2
  x [m] : Inport  Port=3
  vx [m/s] : Inport  Port=4
  Contact! : EnablePort  StatesWhenEnabling=reset
  Data Type Conversion : DataTypeConversion  OutDataTypeStr=double  SaturateOnIntegerOverflow=off  RndMeth=Floor
  Friction Switch : Subsystem
  Gain3 : Gain  Gain=k_gy
  Gain4 : Gain  Gain=1/v_gy_max
  Logical Operator : Logic  Operator=NOT  AllPortsSameDT=off  OutDataTypeStr=boolean
  Mux1 : Mux  Inputs=2
  Sum1 : Sum
  X-Axis Kinetic Friction Model : Subsystem
  X-Axis Static Friction Model : Subsystem
  Y-Axis Ground Force : Fcn  Expr="- u(1)  *  (1-u(2)) * (u(2)<1)"
  Fy_Ground[N] : Outport  OutputWhenDisabled=reset  InitialOutput=0
      settings: AttributesFormatString=initial = '%<InitialOutput>'\nwhen disabled = '%<OutputWhenDisabled>'
  Fx_Friction [N] : Outport  Port=2  OutputWhenDisabled=reset  InitialOutput=0
      settings: AttributesFormatString=initial = '%<InitialOutput>'\nwhen\ndisabled\n'%<OutputWhenDisabled>'
  Stiction! : Outport  Port=3  OutputWhenDisabled=reset  InitialOutput=0
      settings: AttributesFormatString=initial = '%<InitialOutput>'\nwhen\ndisabled\n'%<OutputWhenDisabled>'
  wires:
  Gain4/1 -> Mux1/2
  Gain3/1 -> Mux1/1
  Mux1/1 -> Y-Axis Ground Force/1
  Data Type Conversion/1 -> Stiction!/1
  Logical Operator/1 -> X-Axis Kinetic Friction Model/Enable
  X-Axis Kinetic Friction Model/2(Stiction!) -> Friction Switch/2(Stick!)
  X-Axis Static Friction Model/2(Sliding!) -> Friction Switch/1(Slide!)
  Friction Switch/1(Stiction) -> Data Type Conversion/1, Logical Operator/1, X-Axis Static Friction Model/Enable
  Sum1/1 -> Fx_Friction [N]/1
  X-Axis Static Friction Model/1(F_Stick [N]) -> Sum1/1
  X-Axis Kinetic Friction Model/3(F_Slide [N]) -> Sum1/2
  X-Axis Kinetic Friction Model/1(posFP [m]) -> X-Axis Static Friction Model/4(posFP [m])
  vx [m/s]/1 -> X-Axis Kinetic Friction Model/2(vel [m/s]), X-Axis Static Friction Model/3(vel [m/s])
  x [m]/1 -> X-Axis Kinetic Friction Model/1(pos [m]), X-Axis Static Friction Model/2(pos [m])
  vy [m/s]/1 -> Gain4/1
  dy [m]/1 -> Gain3/1
  Y-Axis Ground Force/1 -> Fy_Ground[N]/1, X-Axis Kinetic Friction Model/3(F_Normal [N]), X-Axis Static Friction Model/1(F_Normal [N])

== system rolling_contact_36_example/36-Point Sliding Contact Model/Body Contact 21/Ground Friction Model ==
  note: Horizontal Ground Friction Model
  note: Vertical Ground Stiction Model
  dy [m] : Inport
  vy [m/s] : Inport  Port=2
  x [m] : Inport  Port=3
  vx [m/s] : Inport  Port=4
  Contact! : EnablePort  StatesWhenEnabling=reset
  Data Type Conversion : DataTypeConversion  OutDataTypeStr=double  SaturateOnIntegerOverflow=off  RndMeth=Floor
  Friction Switch : Subsystem
  Gain3 : Gain  Gain=k_gy
  Gain4 : Gain  Gain=1/v_gy_max
  Logical Operator : Logic  Operator=NOT  AllPortsSameDT=off  OutDataTypeStr=boolean
  Mux1 : Mux  Inputs=2
  Sum1 : Sum
  X-Axis Kinetic Friction Model : Subsystem
  X-Axis Static Friction Model : Subsystem
  Y-Axis Ground Force : Fcn  Expr="- u(1)  *  (1-u(2)) * (u(2)<1)"
  Fy_Ground[N] : Outport  OutputWhenDisabled=reset  InitialOutput=0
      settings: AttributesFormatString=initial = '%<InitialOutput>'\nwhen disabled = '%<OutputWhenDisabled>'
  Fx_Friction [N] : Outport  Port=2  OutputWhenDisabled=reset  InitialOutput=0
      settings: AttributesFormatString=initial = '%<InitialOutput>'\nwhen\ndisabled\n'%<OutputWhenDisabled>'
  Stiction! : Outport  Port=3  OutputWhenDisabled=reset  InitialOutput=0
      settings: AttributesFormatString=initial = '%<InitialOutput>'\nwhen\ndisabled\n'%<OutputWhenDisabled>'
  wires:
  Y-Axis Ground Force/1 -> X-Axis Static Friction Model/1(F_Normal [N]), X-Axis Kinetic Friction Model/3(F_Normal [N]), Fy_Ground[N]/1
  dy [m]/1 -> Gain3/1
  vy [m/s]/1 -> Gain4/1
  x [m]/1 -> X-Axis Static Friction Model/2(pos [m]), X-Axis Kinetic Friction Model/1(pos [m])
  vx [m/s]/1 -> X-Axis Static Friction Model/3(vel [m/s]), X-Axis Kinetic Friction Model/2(vel [m/s])
  X-Axis Kinetic Friction Model/1(posFP [m]) -> X-Axis Static Friction Model/4(posFP [m])
  X-Axis Kinetic Friction Model/3(F_Slide [N]) -> Sum1/2
  X-Axis Static Friction Model/1(F_Stick [N]) -> Sum1/1
  Sum1/1 -> Fx_Friction [N]/1
  Friction Switch/1(Stiction) -> X-Axis Static Friction Model/Enable, Logical Operator/1, Data Type Conversion/1
  X-Axis Static Friction Model/2(Sliding!) -> Friction Switch/1(Slide!)
  X-Axis Kinetic Friction Model/2(Stiction!) -> Friction Switch/2(Stick!)
  Logical Operator/1 -> X-Axis Kinetic Friction Model/Enable
  Data Type Conversion/1 -> Stiction!/1
  Mux1/1 -> Y-Axis Ground Force/1
  Gain3/1 -> Mux1/1
  Gain4/1 -> Mux1/2
